simulink model "PMSM_FOC_R2026a"  (R2026a)
settings: Solver=ode4  StopTime=1  FixedStep=timing_h  MaxStep=1e-6
InitFcn:
  | % Embedded verbatim in the model InitFcn; no helper file is needed to run SLX.
  | teach_model = bdroot;
  | teach_workspace = get_param(teach_model,'ModelWorkspace');
  | teach_cfg_path = [teach_model '/时序设置'];
  | teach_divider = str2double(get_param(teach_cfg_path,'speed_divider'));
  | teach_cycles = str2double(get_param(teach_cfg_path,'pwm_cycles'));
  | validateattributes(teach_divider,{'double'},{'scalar','real','finite','integer','>=',1,'<=',1000});
  | validateattributes(teach_cycles,{'double'},{'scalar','real','finite','integer','>=',1,'<=',20});
  | teach_dt = getVariable(teach_workspace,'dt');
  | teach_period = getVariable(teach_workspace,'Ts_speed');
  | if strcmp(get_param(teach_cfg_path,'speed_on'),'on')
  |     teach_period = teach_dt*teach_divider;
  | end
  | assert(teach_period >= teach_dt && abs(teach_period/teach_dt-round(teach_period/teach_dt))<1e-9, ...
  |     '速度环周期必须为电流控制周期的正整数倍。');
  | teach_names = {'teaching_Ts_speed','teach_pwm_on','teach_pwm_cycles'};
  | teach_values_to_set = {teach_period,double(strcmp(get_param(teach_cfg_path,'pwm_on'),'on')),teach_cycles};
  | for teach_index = 1:numel(teach_names)
  |     if ~isequaln(getVariable(teach_workspace,teach_names{teach_index}),teach_values_to_set{teach_index})
  |         assignin(teach_workspace,teach_names{teach_index},teach_values_to_set{teach_index});
  |     end
  | end
  | 
  | 
  | assignin(get_param(bdroot,'ModelWorkspace'),'decoupling_enabled',double(strcmp(get_param([bdroot '/解耦'],'enabled'),'on')));
  | % Embedded in InitFcn after the pre-existing teaching initialization.
  | tim_m=bdroot;tim_ws=get_param(tim_m,'ModelWorkspace');tim_path=[tim_m '/时序设置'];
  | tim_on=double(strcmp(get_param(tim_path,'real_on'),'on'));
  | tim_period=getVariable(tim_ws,'dt');tim_speed=getVariable(tim_ws,'teaching_Ts_speed');
  | tim_trigger=str2double(get_param(tim_path,'trigger_us'))*1e-6;
  | tim_sync=str2double(get_param(tim_path,'sync_us'))*1e-6;
  | tim_compute=str2double(get_param(tim_path,'compute_us'))*1e-6;
  | tim_guard=str2double(get_param(tim_path,'settle_us'))*1e-6;
  | tim_window=double(strcmp(get_param(tim_path,'window_on'),'on'));
  | tim_hold=double(strcmp(get_param(tim_path,'invalid_hold_on'),'on'));
  | tim_mode=double(strcmp(get_param(tim_path,'update_mode'),'仅谷底（对照）'));
  | tim_h=1e-6;tim_control=tim_period;tim_speed_sample=tim_speed;
  | tim_static=-1;
  | tim_carrier=[0 tim_period/2 0];
  | validateattributes([tim_trigger tim_sync tim_compute tim_guard],{'double'},{'real','finite','nonnegative'});
  | if tim_on
  |  assert(strcmp(get_param(tim_path,'pwm_on'),'off'),'真实时序与旧整周期输出延迟不可同时启用。');
  |  assert(strcmp(get_param([tim_m '/采样设置'],'delay_on'),'off'),'真实时序与旧整周期采样延迟不可同时启用。');
  |  tim_h=62.5e-9;
  |  tim_grid_divider=str2double(get_param(tim_path,'grid_divider'));
  |  validateattributes(tim_grid_divider,{'double'},{'scalar','integer','>=',1,'<=',2});
  |  % Optional finer grid for convergence checks, still configured explicitly.
  |  tim_h=tim_h/tim_grid_divider;
  |  validateattributes(tim_h,{'double'},{'scalar','finite','positive'});
  |  tim_jeos=tim_trigger+tim_sync+4.5e-6;
  |  assert(tim_compute>=tim_h,'计算耗时至少为一个事件网格，避免写入读取同拍未完成指令。');
  |  assert(tim_jeos+tim_compute<tim_period,'本版要求整组转换及计算在同一PWM周期内完成。');
  |  assert(tim_jeos>0 && tim_jeos<tim_period);
  |  timing_grid_values=[tim_trigger tim_sync tim_compute tim_guard 1.1875e-6 1.5e-6 tim_period tim_speed];
  |  assert(all(abs(timing_grid_values/tim_h-round(timing_grid_values/tim_h))<1e-7),'事件时间必须落在62.5ns（或更细）网格上。');
  |  tim_control=[tim_period tim_jeos];
  |  tim_static=0;
  |  tim_speed_sample=[tim_speed tim_jeos+tim_speed-tim_period];
  |  % Existing comparator is carrier>=threshold; inverted carrier implements PWM1.
  |  tim_carrier=[tim_period/2 0 tim_period/2];
  | ... (+37 lines)
model workspace (MATLAB code in the model file):
  | % Embedded reference for the CHENSHA 200W nominal firmware profile.
  | % Source: AxDr_L dev 48d6e86814ac6657b1313b4c92ef24c88f492e07,
  | % User/config/motor_config.h. Not a measured plant identification.
  | % This script is embedded into the SLX Model Workspace; no path dependency.
  | T=1e-6; % Numerical step [s]; switching detail remains ideal/average equivalent
  | MotorProfile='CHENSHA 200W / firmware profile revision 2';
  | MotorSourceCommit='48d6e86814ac6657b1313b4c92ef24c88f492e07';
  | Pn=200; % Nameplate power [W], stored as specified; not forced to equal Tn*wm
  | Un=24; Vdc=24;
  | I_rated_rms=11.5; % Phase RMS [A], nameplate
  | I_peak_rms=23; % Phase RMS [A], nameplate peak
  | In=sqrt(2)*I_rated_rms; % Phase amplitude / dq nominal current [A]
  | I_peak=sqrt(2)*I_peak_rms; % Phase amplitude [A]
  | n=3000; % Speed reference and nominal speed [rpm]
  | p=5; % Pole pairs
  | Rs=0.105125; % Phase resistance [ohm], firmware profile convention
  | Ld=103.7615e-6; Lq=103.7615e-6; Ls=Ld; % dq inductance [H]
  | phis=0.06/(sqrt(2)*1.5*p); % Flux [Wb], derived from Kt_rms; Ke definition pending
  | J=32e-6; % Rotor inertia [kg*m^2], profile value; coupled inertia not identified
  | F=0; % Firmware profile placeholder; does not prove physical friction is zero
  | Kt=1.5*p*phis; % Torque per dq amplitude [N*m/A]
  | Tn=0.69; T_peak=1.38; % Nameplate torque [N*m]
  | Iq_limit=8; % Firmware bench command limit [A], not RMS nameplate current
  | accel_limit_rad_s2=1200; % Stored only; a command ramp is not implemented here
  | speed_peak_rad_s=335; % Stored only; speed protection is not implemented here
  | I_protection_A=10; Vbus_protection_high_V=30; Vbus_protection_low_V=10;
  | % Protection values above are references, not active trip logic in this model.
  | RE=10000; rr=2*pi/RE; % Mechanical counts/revolution; ABZ estimator not implemented
  | encoder_direction=-1; % Stored firmware setting; ideal plant angle stays unchanged
  | fN=p*n/60; wN=2*pi*fN;
  | ki_p=0.8; ki_i=1; % Original unused/auxiliary constants retained
  | fc=20e3; Ts=1/fc; dt=Ts;
  | Ts_speed=2*dt; % Base speed task 10kHz; current/PWM 20kHz
  | w_sb=2*pi*fN*1.2;
  | fcb=1000; fwb=50; wc=2*pi*fcb; wsc=2*pi*fwb;
  | % fcb/fwb describe the previous gain design, not measured bandwidth of this motor.
  | K=30/pi; % Mechanical rad/s to rpm
  | % PI_GAINS_FROZEN: inserted from the validated previous workspace, bit-for-bit.
  | kp_w=0.00069087230807625508;
  | ki_w=0.04340878735241975;
  | ks_w=0.98718608264211138;
  | kp_id=0.7539822368615503;
  | ki_id=879.64594300514204;
  | ks_id=1.1309733552923253;
  | kp_iq=0.7539822368615503;
  | ki_iq=879.64594300514204;
  | ks_iq=1.1309733552923253;
  | Bm=0;
  | uplimit_w=Kt*Iq_limit; downlimit_w=-uplimit_w; % Speed PI output is torque [N*m]
  | % Ld=Lq and id_ref=0, so Te_ref/Kt is exactly the iq demand before dynamics.
  | uplimit_id=Vdc/sqrt(3); downlimit_id=-uplimit_id;
  | uplimit_iq=Vdc/sqrt(3); downlimit_iq=-uplimit_iq;
  | teaching_Ts_speed=Ts_speed; teach_pwm_on=0; teach_pwm_cycles=1;
  | 
  | decoupling_enabled=1; voltage_utilization=0.96; % Algorithm stage 2; PI gains frozen
  | 
  | timing_on=0; timing_h=1e-6; timing_control_sample=dt; timing_speed_sample=Ts_speed; timing_static_math=-1;
  | timing_carrier_y=[0 Ts/2 0];
  | timing_adc_cfg=[0 0 0 1e-6 Ts 24.375e-6 1.1875e-6 1.5e-6 0 .5e-6 2];
  | timing_pwm_cfg=[0 1e-6 Ts 24.375e-6 1.1875e-6 1.5e-6 0 5e-6 0 4000];
  | 
  | dead_gate_on=0; dead_h=1e-6; dead_gate_cfg=[0 1e-6 .5e-6];
  | dead_comp_cfg=[0 .5e-6 Ts .05]; dead_bridge_cfg=[p phis .01 0 .01 .7];
undefined symbols (not defined in the file or in its folder): DiscIntNeverNeededParam
libraries: simulink x3
(part 2 of 2)

== system PMSM_FOC_R2026a/功率观测 ==
  note: 01 理想相电压 [V]
  note: 02 实际相电压 [V]
  note: 03 平均压降 [V]
  实际相电压 : Scope
      settings: SampleTime=T  Title=实际相电压 [V]
  平均压降 : Scope
      settings: SampleTime=dt  Title=平均压降 [V]
  总览 : Scope  NumInputPorts=8
      settings: SampleTime=T  TimeSpan=0.12  ActiveDisplayString=8  Title=dq补偿 [V]
  极性保留 : Terminator
  理想相电压 : Scope
      settings: SampleTime=T  Title=理想相电压 [V]
  真实电流保留 : Terminator
  续流分组 : Demux  Outputs=[3 3 3]
  补偿分组 : Demux  Outputs=[3 2 3]
  wires:
  [ObsPhaseIdeal] -> 理想相电压/1, 总览/1
  [ObsPhaseActual] -> 实际相电压/1, 总览/2
  [ObsPowerDrop] -> 平均压降/1, 总览/3
  [ObsFreewheel] -> 续流分组/1
  续流分组/3 -> 真实电流保留/1
  [ObsDeadComp] -> 补偿分组/1
  补偿分组/3 -> 极性保留/1
  [SWact] -> 总览/4
  续流分组/1 -> 总览/5
  续流分组/2 -> 总览/6
  补偿分组/1 -> 总览/7
  补偿分组/2 -> 总览/8

== system PMSM_FOC_R2026a/功率设置 ==
  三相压降 : Mux  Inputs=3
  压降1 : Fcn  Expr=dead_on*dead_us*1e-6/Ts*(u(4)+drop_on*vf)*u(1)/(abs(u(1))+blend_A)+drop_on*ron*u(1)
  压降2 : Fcn  Expr=dead_on*dead_us*1e-6/Ts*(u(4)+drop_on*vf)*u(2)/(abs(u(2))+blend_A)+drop_on*ron*u(2)
  压降3 : Fcn  Expr=dead_on*dead_us*1e-6/Ts*(u(4)+drop_on*vf)*u(3)/(abs(u(3))+blend_A)+drop_on*ron*u(3)
  去共模 : Gain  Gain=eye(3)-ones(3)/3  Multiplication=Matrix(K*u)
  启用 : Constant  Value=(~dead_gate_on)&&(dead_on||drop_on)
  周期电流 : ZeroOrderHold  SampleTime=Ts
  记录_obs_power_drop : ToWorkspace  VariableName=obs_power_drop  SaveFormat=Timeseries  SampleTime=timing_control_sample
  输入 : Mux  Inputs=2
  tag scope: ObsPowerDrop=global, ObsPowerOn=global
  wires:
  [Currentabc] -> 周期电流/1
  周期电流/1 -> 输入/1
  [UDC] -> 输入/2
  输入/1 -> 压降1/1, 压降2/1, 压降3/1
  压降1/1 -> 三相压降/1
  压降2/1 -> 三相压降/2
  压降3/1 -> 三相压降/3
  三相压降/1 -> 去共模/1
  去共模/1 -> [ObsPowerDrop], 记录_obs_power_drop/1
  启用/1 -> [ObsPowerOn]

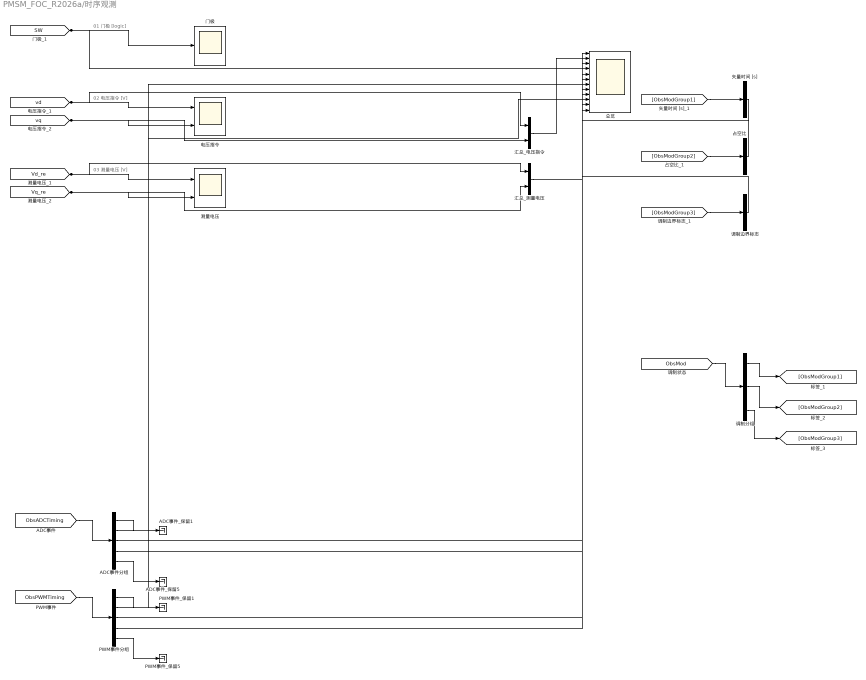
== system PMSM_FOC_R2026a/时序观测 ==
  note: 01 门极 [logic]
  note: 02 电压指令 [V]
  note: 03 测量电压 [V]
  ADC事件_保留1 : Terminator
  ADC事件_保留5 : Terminator
  ADC事件分组 : Demux  Outputs=[1 5 3 4 2]
  PWM事件_保留1 : Terminator
  PWM事件_保留5 : Terminator
  PWM事件分组 : Demux  Outputs=[2 3 3 1 3]
  占空比 : Mux  Inputs=1
  总览 : Scope  NumInputPorts=12
      settings: SampleTime=T  TimeSpan=0.12  ActiveDisplayString=12  Title=采样至生效 [s]
  汇总_测量电压 : Mux  Inputs=2
  汇总_电压指令 : Mux  Inputs=2
  测量电压 : Scope  NumInputPorts=2
      settings: SampleTime=T  Title=测量电压 [V]
  电压指令 : Scope  NumInputPorts=2
      settings: SampleTime=dt  Title=电压指令 [V]
  矢量时间 [s] : Mux  Inputs=1
  调制分组 : Demux  Outputs=[3 3 2]
  调制边界标志 : Mux  Inputs=1
  门极 : Scope
      settings: SampleTime=T  Title=门极 [logic]
  wires:
  [SW] -> 门极/1, 总览/1
  [vd] -> 电压指令/1, 汇总_电压指令/1
  [vq] -> 电压指令/2, 汇总_电压指令/2
  [Vd_re] -> 测量电压/1, 汇总_测量电压/1
  [Vq_re] -> 测量电压/2, 汇总_测量电压/2
  汇总_电压指令/1 -> 总览/2
  汇总_测量电压/1 -> 总览/3
  [ObsMod] -> 调制分组/1
  调制分组/1 -> [ObsModGroup1]
  调制分组/2 -> [ObsModGroup2]
  调制分组/3 -> [ObsModGroup3]
  [ObsModGroup1] -> 矢量时间 [s]/1
  矢量时间 [s]/1 -> 总览/4
  [ObsModGroup2] -> 占空比/1
  占空比/1 -> 总览/5
  [ObsModGroup3] -> 调制边界标志/1
  调制边界标志/1 -> 总览/6
  [ObsADCTiming] -> ADC事件分组/1
  ADC事件分组/1 -> ADC事件_保留1/1
  ADC事件分组/5 -> ADC事件_保留5/1
  [ObsPWMTiming] -> PWM事件分组/1
  PWM事件分组/1 -> PWM事件_保留1/1
  PWM事件分组/5 -> PWM事件_保留5/1
  ADC事件分组/2 -> 总览/7
  ADC事件分组/3 -> 总览/8
  ADC事件分组/4 -> 总览/9
  PWM事件分组/2 -> 总览/10
  PWM事件分组/3 -> 总览/11
  PWM事件分组/4 -> 总览/12

== system PMSM_FOC_R2026a/时序设置 ==

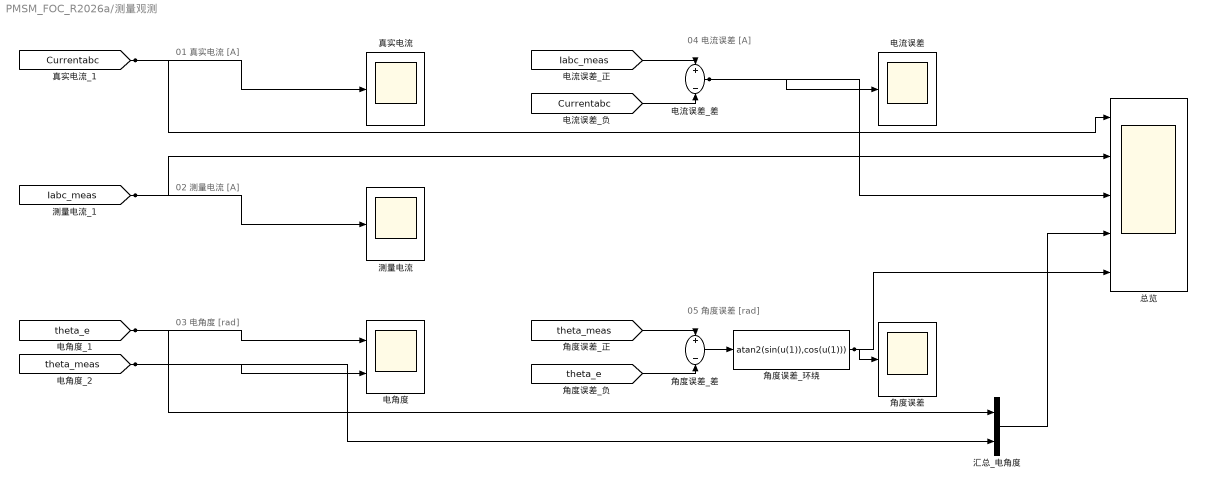
== system PMSM_FOC_R2026a/测量观测 ==
  note: 01 真实电流 [A]
  note: 02 测量电流 [A]
  note: 03 电角度 [rad]
  note: 04 电流误差 [A]
  note: 05 角度误差 [rad]
  总览 : Scope  NumInputPorts=5
      settings: SampleTime=dt  TimeSpan=0.12  ActiveDisplayString=5  Title=角度误差 [rad]
  汇总_电角度 : Mux  Inputs=2
  测量电流 : Scope
      settings: SampleTime=dt  Title=测量电流 [A]
  电流误差 : Scope
      settings: SampleTime=dt  Title=电流误差 [A]
  电流误差_差 : Sum  Inputs=+-
  电角度 : Scope  NumInputPorts=2
      settings: SampleTime=dt  Title=电角度 [rad]
  真实电流 : Scope
      settings: SampleTime=dt  Title=真实电流 [A]
  角度误差 : Scope
      settings: SampleTime=dt  Title=角度误差 [rad]
  角度误差_差 : Sum  Inputs=+-
  角度误差_环绕 : Fcn  Expr=atan2(sin(u(1)),cos(u(1)))
  wires:
  [Currentabc] -> 真实电流/1, 总览/1
  [Iabc_meas] -> 测量电流/1, 总览/2
  [theta_e] -> 电角度/1, 汇总_电角度/1
  [theta_meas] -> 电角度/2, 汇总_电角度/2
  [Iabc_meas] -> 电流误差_差/1
  [Currentabc] -> 电流误差_差/2
  电流误差_差/1 -> 电流误差/1, 总览/3
  [theta_meas] -> 角度误差_差/1
  [theta_e] -> 角度误差_差/2
  角度误差_差/1 -> 角度误差_环绕/1
  角度误差_环绕/1 -> 角度误差/1, 总览/5
  汇总_电角度/1 -> 总览/4

== system PMSM_FOC_R2026a/角度设置 ==
  传递延迟 : Delay  DelayLength=delay_cycles  InitialCondition=0  SampleTime=timing_control_sample
  偏置 : Constant  Value=bias_on*bias_deg*pi/180
  偏置求和 : Sum
  启用 : Constant  Value=bias_on||quant_on||delay_on
  延迟开关 : Constant  Value=delay_on
  延迟选择 : Switch  Criteria=u2 ~= 0  SaturateOnIntegerOverflow=off  InputSameDT=off
  总选择 : Switch  Criteria=u2 ~= 0  SaturateOnIntegerOverflow=off  InputSameDT=off
  最短角差 : Fcn  Expr=atan2(sin(u(1)),cos(u(1)))
  角度差 : Sum  Inputs=+-
  角度环绕 : Fcn  Expr=u(1)-2*pi*floor(u(1)/(2*pi))
  记录_log_theta_error : ToWorkspace  VariableName=log_theta_error  SaveFormat=Timeseries  SampleTime=timing_control_sample
  记录_log_theta_meas : ToWorkspace  VariableName=log_theta_meas  SaveFormat=Timeseries  SampleTime=timing_control_sample
  记录_log_theta_true : ToWorkspace  VariableName=log_theta_true  SaveFormat=Timeseries  SampleTime=timing_control_sample
  量化 : Quantizer  QuantizationInterval=step_deg*pi/180
  量化开关 : Constant  Value=quant_on
  量化选择 : Switch  Criteria=u2 ~= 0  SaturateOnIntegerOverflow=off  InputSameDT=off
  tag scope: theta_meas=global
  wires:
  [theta_e] -> 偏置求和/1, 总选择/3, 角度差/2, 记录_log_theta_true/1
  偏置/1 -> 偏置求和/2
  偏置求和/1 -> 量化/1, 量化选择/3
  量化/1 -> 量化选择/1
  量化开关/1 -> 量化选择/2
  量化选择/1 -> 角度环绕/1
  角度环绕/1 -> 传递延迟/1, 延迟选择/3
  传递延迟/1 -> 延迟选择/1
  延迟开关/1 -> 延迟选择/2
  延迟选择/1 -> 总选择/1
  启用/1 -> 总选择/2
  总选择/1 -> [theta_meas], 角度差/1, 记录_log_theta_meas/1
  角度差/1 -> 最短角差/1
  最短角差/1 -> 记录_log_theta_error/1

== system PMSM_FOC_R2026a/解耦 ==

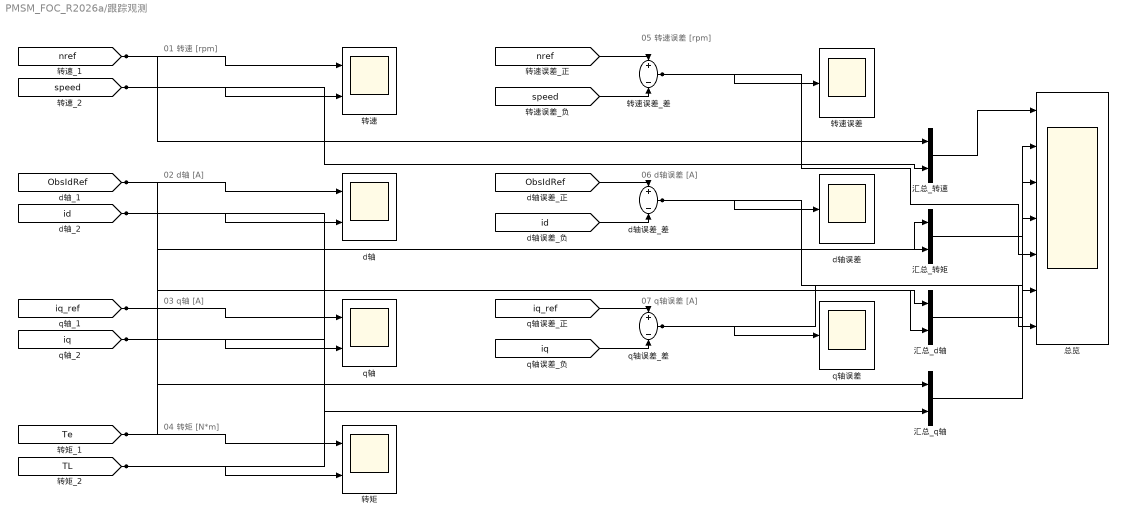
== system PMSM_FOC_R2026a/跟踪观测 ==
  note: 01 转速 [rpm]
  note: 02 d轴 [A]
  note: 03 q轴 [A]
  note: 04 转矩 [N*m]
  note: 05 转速误差 [rpm]
  note: 06 d轴误差 [A]
  note: 07 q轴误差 [A]
  d轴 : Scope  NumInputPorts=2
      settings: SampleTime=dt  Title=d轴 [A]
  d轴误差 : Scope
      settings: SampleTime=dt  Title=d轴误差 [A]
  d轴误差_差 : Sum  Inputs=+-
  q轴 : Scope  NumInputPorts=2
      settings: SampleTime=dt  Title=q轴 [A]
  q轴误差 : Scope
      settings: SampleTime=dt  Title=q轴误差 [A]
  q轴误差_差 : Sum  Inputs=+-
  总览 : Scope  NumInputPorts=7
      settings: SampleTime=dt  TimeSpan=0.12  ActiveDisplayString=7  Title=q轴误差 [A]
  汇总_d轴 : Mux  Inputs=2
  汇总_q轴 : Mux  Inputs=2
  汇总_转矩 : Mux  Inputs=2
  汇总_转速 : Mux  Inputs=2
  转矩 : Scope  NumInputPorts=2
      settings: SampleTime=dt  Title=转矩 [N*m]
  转速 : Scope  NumInputPorts=2
      settings: SampleTime=dt  Title=转速 [rpm]
  转速误差 : Scope
      settings: SampleTime=dt  Title=转速误差 [rpm]
  转速误差_差 : Sum  Inputs=+-
  wires:
  [nref] -> 转速/1, 汇总_转速/1
  [speed] -> 转速/2, 汇总_转速/2
  [ObsIdRef] -> d轴/1, 汇总_d轴/1
  [id] -> d轴/2, 汇总_d轴/2
  [iq_ref] -> q轴/1, 汇总_q轴/1
  [iq] -> q轴/2, 汇总_q轴/2
  [Te] -> 转矩/1, 汇总_转矩/1
  [TL] -> 转矩/2, 汇总_转矩/2
  [nref] -> 转速误差_差/1
  [speed] -> 转速误差_差/2
  转速误差_差/1 -> 转速误差/1, 总览/5
  [ObsIdRef] -> d轴误差_差/1
  [id] -> d轴误差_差/2
  d轴误差_差/1 -> d轴误差/1, 总览/6
  [iq_ref] -> q轴误差_差/1
  [iq] -> q轴误差_差/2
  q轴误差_差/1 -> q轴误差/1, 总览/7
  汇总_转速/1 -> 总览/1
  汇总_转矩/1 -> 总览/2
  汇总_d轴/1 -> 总览/3
  汇总_q轴/1 -> 总览/4

== system PMSM_FOC_R2026a/输出延迟 ==
  指令 : Inport
  CCR预装载 : MATLAB Function  TreatAsAtomicUnit=on
  事件时钟 : DigitalClock  SampleTime=timing_h
  启用 : Constant  Value=teach_pwm_on
  周期延迟 : Delay  DelayLength=teach_pwm_cycles  InitialCondition=0  SampleTime=timing_control_sample
  指令缓存 : UnitDelay  InitialCondition=Ts/4  SampleTime=timing_h
  时序参数 : Constant  Value=timing_pwm_cfg
  记录_log_Tcm_applied : ToWorkspace  VariableName=log_Tcm_applied  SaveFormat=Timeseries  SampleTime=timing_control_sample
  记录_log_Tcm_requested : ToWorkspace  VariableName=log_Tcm_requested  SaveFormat=Timeseries  SampleTime=timing_control_sample
  记录_obs_pwm_timing : ToWorkspace  VariableName=obs_pwm_timing  SaveFormat=Timeseries  SampleTime=timing_h
  输出方式 : VariantSource  VariantControls={real_mode==1, real_mode==0}
  选择 : Switch  Criteria=u2 ~= 0  SaturateOnIntegerOverflow=off  InputSameDT=off
  阈值向量 : Reshape
  生效 : Outport
  tag scope: ObsPWMTiming=global
  wires:
  指令/1 -> 周期延迟/1, 选择/3, 记录_log_Tcm_requested/1, 指令缓存/1
  周期延迟/1 -> 选择/1
  启用/1 -> 选择/2
  选择/1 -> 输出方式/2
  事件时钟/1 -> CCR预装载/1(t)
  时序参数/1 -> CCR预装载/3(cfg)
  指令缓存/1 -> CCR预装载/2(request)
  CCR预装载/1(applied) -> 阈值向量/1
  输出方式/1 -> 生效/1, 记录_log_Tcm_applied/1
  阈值向量/1 -> 输出方式/1
  CCR预装载/2(diag) -> 记录_obs_pwm_timing/1, [ObsPWMTiming]

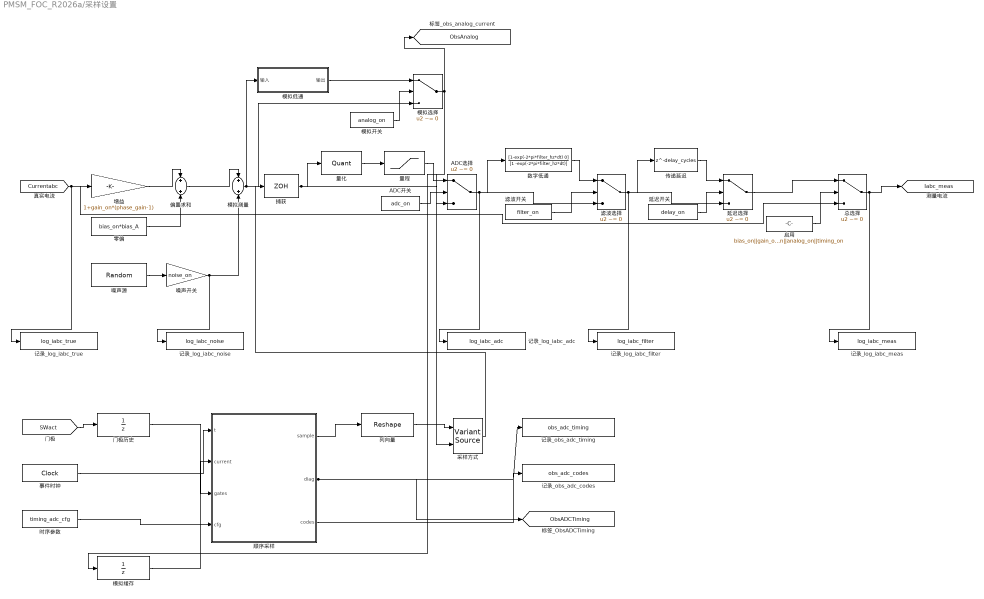
== system PMSM_FOC_R2026a/采样设置 ==
  ADC开关 : Constant  Value=adc_on
  ADC选择 : Switch  Criteria=u2 ~= 0  SaturateOnIntegerOverflow=off  InputSameDT=off
  事件时钟 : DigitalClock  SampleTime=timing_h
  传递延迟 : Delay  DelayLength=delay_cycles  InitialCondition=0  SampleTime=timing_control_sample
  偏置求和 : Sum
  列向量 : Reshape  OutputDimensionality=Column vector (2-D)
  启用 : Constant  Value=bias_on||gain_on||noise_on||adc_on||filter_on||delay_on||analog_on||timing_on
  噪声开关 : Gain  Gain=noise_on
  噪声源 : RandomNumber  Mean=[0 0 0]  Variance=noise_rms^2  Seed=noise_seed+[0 1 2]  SampleTime=timing_control_sample
  增益 : Gain  Gain=1+gain_on*(phase_gain-1)
  延迟开关 : Constant  Value=delay_on
  延迟选择 : Switch  Criteria=u2 ~= 0  SaturateOnIntegerOverflow=off  InputSameDT=off
  总选择 : Switch  Criteria=u2 ~= 0  SaturateOnIntegerOverflow=off  InputSameDT=off
  捕获 : ZeroOrderHold  SampleTime=timing_control_sample
  数字低通 : DiscreteTransferFcn  Numerator=[1-exp(-2*pi*filter_hz*dt) 0]  Denominator=[1 -exp(-2*pi*filter_hz*dt)]  SampleTime=timing_control_sample
  时序参数 : Constant  Value=timing_adc_cfg
  模拟低通 : Subsystem
  模拟开关 : Constant  Value=analog_on
  模拟测量 : Sum
  模拟缓存 : UnitDelay  InitialCondition=[0;0;0]  SampleTime=timing_h
  模拟选择 : Switch  Criteria=u2 ~= 0  SaturateOnIntegerOverflow=off  InputSameDT=off
  滤波开关 : Constant  Value=filter_on
  滤波选择 : Switch  Criteria=u2 ~= 0  SaturateOnIntegerOverflow=off  InputSameDT=off
  记录_log_iabc_adc : ToWorkspace  VariableName=log_iabc_adc  SaveFormat=Timeseries  SampleTime=timing_control_sample
  记录_log_iabc_filter : ToWorkspace  VariableName=log_iabc_filter  SaveFormat=Timeseries  SampleTime=timing_control_sample
  记录_log_iabc_meas : ToWorkspace  VariableName=log_iabc_meas  SaveFormat=Timeseries  SampleTime=timing_control_sample
  记录_log_iabc_noise : ToWorkspace  VariableName=log_iabc_noise  SaveFormat=Timeseries  SampleTime=timing_control_sample
  记录_log_iabc_true : ToWorkspace  VariableName=log_iabc_true  SaveFormat=Timeseries  SampleTime=timing_control_sample
  记录_obs_adc_codes : ToWorkspace  VariableName=obs_adc_codes  SaveFormat=Timeseries  SampleTime=timing_control_sample
  记录_obs_adc_timing : ToWorkspace  VariableName=obs_adc_timing  SaveFormat=Timeseries  SampleTime=timing_h
  采样方式 : VariantSource  VariantControls={real_mode==1, real_mode==0}
  量化 : Quantizer  QuantizationInterval=2*adc_span/2^adc_bits
  量程 : Saturate  UpperLimit=adc_span-2*adc_span/2^adc_bits  LowerLimit=-adc_span
  门极历史 : UnitDelay  InitialCondition=[0 1 0 1 0 1]  SampleTime=timing_h
  零偏 : Constant  Value=bias_on*bias_A
  顺序采样 : MATLAB Function  TreatAsAtomicUnit=on
  tag scope: Iabc_meas=global, ObsADCTiming=global, ObsAnalog=global
  wires:
  [Currentabc] -> 增益/1, 总选择/3, 记录_log_iabc_true/1
  增益/1 -> 偏置求和/1
  零偏/1 -> 偏置求和/2
  偏置求和/1 -> 模拟测量/1
  噪声源/1 -> 噪声开关/1
  噪声开关/1 -> 模拟测量/2, 记录_log_iabc_noise/1
  捕获/1 -> 量化/1, ADC选择/3
  量化/1 -> 量程/1
  量程/1 -> ADC选择/1
  ADC开关/1 -> ADC选择/2
  ADC选择/1 -> 数字低通/1, 滤波选择/3, 记录_log_iabc_adc/1
  数字低通/1 -> 滤波选择/1
  滤波开关/1 -> 滤波选择/2
  滤波选择/1 -> 传递延迟/1, 延迟选择/3, 记录_log_iabc_filter/1
  传递延迟/1 -> 延迟选择/1
  延迟开关/1 -> 延迟选择/2
  延迟选择/1 -> 总选择/1
  启用/1 -> 总选择/2
  总选择/1 -> [Iabc_meas], 记录_log_iabc_meas/1
  模拟测量/1 -> 模拟低通/1(输入), 模拟选择/3
  模拟低通/1(输出) -> 模拟选择/1
  模拟开关/1 -> 模拟选择/2
  模拟选择/1 -> [ObsAnalog], 模拟缓存/1, 采样方式/2
  [SWact] -> 门极历史/1
  事件时钟/1 -> 顺序采样/1(t)
  门极历史/1 -> 顺序采样/3(gates)
  时序参数/1 -> 顺序采样/4(cfg)
  模拟缓存/1 -> 顺序采样/2(current)
  顺序采样/1(sample) -> 列向量/1
  采样方式/1 -> 捕获/1
  列向量/1 -> 采样方式/1
  顺序采样/2(diag) -> 记录_obs_adc_timing/1, [ObsADCTiming]
  顺序采样/3(codes) -> 记录_obs_adc_codes/1

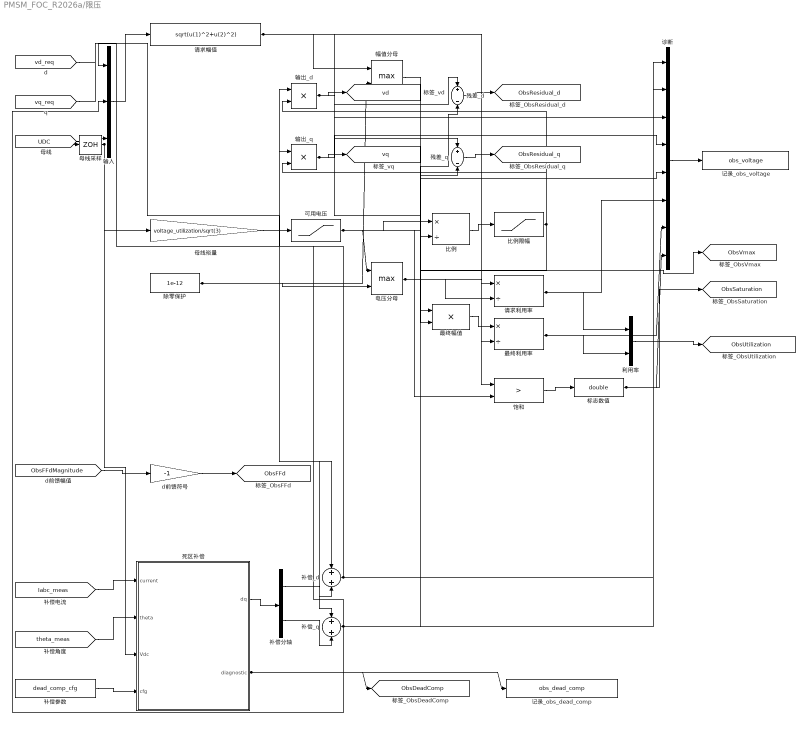
== system PMSM_FOC_R2026a/限压 ==
  d前馈符号 : Gain  Gain=-1
  利用率 : Mux  Inputs=2
  可用电压 : Saturate  UpperLimit=inf  LowerLimit=0
  幅值分母 : MinMax  Function=max  Inputs=2
  最终利用率 : Product  Inputs=*/
  最终幅值 : Product
  标志数值 : DataTypeConversion  OutDataTypeStr=double  SaturateOnIntegerOverflow=off  RndMeth=Floor
  死区补偿 : MATLAB Function  TreatAsAtomicUnit=on
  残差_d : Sum  Inputs=+-
  残差_q : Sum  Inputs=+-
  母线裕量 : Gain  Gain=voltage_utilization/sqrt(3)
  母线采样 : ZeroOrderHold  SampleTime=timing_control_sample
  比例 : Product  Inputs=*/
  比例限幅 : Saturate  UpperLimit=1  LowerLimit=0
  电压分母 : MinMax  Function=max  Inputs=2
  补偿_d : Sum
  补偿_q : Sum
  补偿分轴 : Demux  Outputs=2
  补偿参数 : Constant  Value=dead_comp_cfg
  记录_obs_dead_comp : ToWorkspace  VariableName=obs_dead_comp  SaveFormat=Timeseries  SampleTime=timing_control_sample
  记录_obs_voltage : ToWorkspace  VariableName=obs_voltage  SaveFormat=Timeseries  SampleTime=timing_control_sample
  诊断 : Mux  Inputs=8
  请求利用率 : Product  Inputs=*/
  请求幅值 : Fcn  Expr=sqrt(u(1)^2+u(2)^2)
  输入 : Mux  Inputs=3
  输出_d : Product
  输出_q : Product
  除零保护 : Constant  Value=1e-12
  饱和 : RelationalOperator  Operator=>  OutDataTypeStr=boolean  RndMeth=Simplest  InputSameDT=off
  tag scope: ObsDeadComp=global, ObsFFd=global, ObsResidual_d=global, ObsResidual_q=global, ObsSaturation=global, ObsUtilization=global, ObsVmax=global, vd=global, vq=global
  wires:
  [UDC] -> 母线采样/1
  [vd_req] -> 补偿_d/1
  [vq_req] -> 补偿_q/1
  母线采样/1 -> 输入/3, 母线裕量/1, 死区补偿/3(Vdc)
  输入/1 -> 请求幅值/1
  母线裕量/1 -> 可用电压/1
  请求幅值/1 -> 幅值分母/1, 请求利用率/1, 最终幅值/1, 饱和/1
  除零保护/1 -> 幅值分母/2, 电压分母/2
  可用电压/1 -> 电压分母/1, 比例/1, 诊断/5, 饱和/2, [ObsVmax]
  幅值分母/1 -> 比例/2
  比例/1 -> 比例限幅/1
  比例限幅/1 -> 输出_d/2, 输出_q/2, 最终幅值/2
  输出_d/1 -> [vd], 残差_d/1, 诊断/3
  残差_d/1 -> [ObsResidual_d]
  输出_q/1 -> [vq], 残差_q/1, 诊断/4
  残差_q/1 -> [ObsResidual_q]
  电压分母/1 -> 请求利用率/2, 最终利用率/2
  请求利用率/1 -> 诊断/6, 利用率/1
  最终幅值/1 -> 最终利用率/1
  最终利用率/1 -> 诊断/7, 利用率/2
  饱和/1 -> 标志数值/1
  标志数值/1 -> 诊断/8, [ObsSaturation]
  诊断/1 -> 记录_obs_voltage/1
  利用率/1 -> [ObsUtilization]
  [ObsFFdMagnitude] -> d前馈符号/1
  d前馈符号/1 -> [ObsFFd]
  [Iabc_meas] -> 死区补偿/1(current)
  [theta_meas] -> 死区补偿/2(theta)
  补偿参数/1 -> 死区补偿/4(cfg)
  死区补偿/1(dq) -> 补偿分轴/1
  补偿分轴/1 -> 补偿_d/2
  补偿_d/1 -> 输入/1, 输出_d/1, 残差_d/2, 诊断/1
  补偿分轴/2 -> 补偿_q/2
  补偿_q/1 -> 输入/2, 输出_q/1, 残差_q/2, 诊断/2
  死区补偿/2(diagnostic) -> [ObsDeadComp], 记录_obs_dead_comp/1

== system PMSM_FOC_R2026a/采样设置/模拟低通 ==
  输入 : Inport
  RC1 : TransferFcn  Numerator=[2*pi*analog_hz]  Denominator=[1 2*pi*analog_hz]
  RC2 : TransferFcn  Numerator=[2*pi*analog_hz]  Denominator=[1 2*pi*analog_hz]
  RC3 : TransferFcn  Numerator=[2*pi*analog_hz]  Denominator=[1 2*pi*analog_hz]
  分相 : Demux  Outputs=3
  合相 : Mux  Inputs=3
  输出 : Outport
  wires:
  输入/1 -> 分相/1
  合相/1 -> 输出/1
  分相/1 -> RC1/1
  RC1/1 -> 合相/1
  分相/2 -> RC2/1
  RC2/1 -> 合相/2
  分相/3 -> RC3/1
  RC3/1 -> 合相/3

== matlab function PMSM_FOC_R2026a/采样设置/顺序采样 ==
  settings: updateMethod=DISCRETE  sampleTime=timing_h
  data: t input; sample output size=[1 3]; current input; gates input; cfg input; diag output size=[1 15]; codes output size=[1 3]
function [sample,diag,codes] = timing_adc(t,current,gates,cfg)
%#codegen
% cfg: on, window, hold-invalid, h, Ts, trigger, aperture, rank, sync, guard, speed divider.
% Quantized event grid; outputs are published together at JEOS, in A/B/C order.
persistent captured delivered valid elapsed aperture_ok last_good raw_codes
if isempty(captured)
 captured=zeros(1,3);delivered=zeros(1,3);valid=zeros(1,3);
 elapsed=zeros(1,3);aperture_ok=ones(1,3);last_good=zeros(1,3);raw_codes=2048*ones(1,3);
end
sample=delivered;codes=raw_codes;diag=zeros(1,15);
if cfg(1)==0,return;end
h=cfg(4);N=round(cfg(5)/h);tick=round(t/h);phase=mod(tick,N);
tr=round((cfg(6)+cfg(9))/h);ap=round(cfg(7)/h);rank=round(cfg(8)/h);
guard=ceil(cfg(10)/h);pulse=zeros(1,5);
if phase==tr,pulse(1)=1;end
for k=1:3
 % Gates are sampled one grid tick earlier to avoid an algebraic gate loop.
 if gates(2*k)>0.5,elapsed(k)=elapsed(k)+1;else,elapsed(k)=0;end
 r=3-k;start=tr+r*rank;finish=start+ap;
 if phase==start,aperture_ok(k)=double(elapsed(k)>guard);end
 if phase>=start && phase<=finish && elapsed(k)<=guard,aperture_ok(k)=0;end
 if phase==finish
  valid(k)=aperture_ok(k);pulse(r+2)=1;
 end
 % Input read buffer is one tick old. Read on the following tick so the
 % captured physical value remains exactly at the aperture endpoint.
 if phase==finish+1
  captured(k)=current(k);
  % Low-side OFF has no phase-current observation. Zero is an explicit
  % teaching approximation, not a calibrated amplifier switching transient.
  if cfg(2)>0 && valid(k)==0,captured(k)=0;end
  if valid(k)>0,last_good(k)=captured(k);end
  if cfg(2)>0 && cfg(3)>0 && valid(k)==0,captured(k)=last_good(k);end
 end
end
jeos=tr+3*rank;
if phase==jeos
 delivered=captured;raw_codes=min(4095,max(0,round(2048+captured/(165/4096))));pulse(5)=1;
end
sample=delivered;codes=raw_codes;
% Phase, trigger, C/B/A hold pulses, JEOS, validity ABC, sampled ABC, sum.
diag=[phase*h pulse(1:4) pulse(5) valid delivered sum(delivered) ...
       double(mod(floor(tick/N),cfg(11))==cfg(11)-1 && phase==jeos) double(phase==jeos)];
end

== matlab function PMSM_FOC_R2026a/SVPWM Function v1.0 ==
  data: alpha input; beta input; Vdc input; Ts input; Tcm output; sector output; diagnostic output
function [Tcm,sector,diagnostic] = fcn(alpha,beta,Vdc,Ts)
% Original six-sector construction, with simultaneous overmodulation scaling.
% Tcm is a threshold in [0,Ts/2]; upper duty = 1-2*Tcm/Ts.
% diagnostic: t1,t2,total zero-vector time,Da,Db,Dc,overmodulated,bounds_guard.
Tcm=ones(1,3)*Ts/4;sector=0;
diagnostic=[0 0 Ts .5 .5 .5 0 0];
if Vdc<=0 || Ts<=0 || (alpha==0 && beta==0),return;end
ref1=beta;ref2=(-beta+sqrt(3)*alpha)/2;ref3=(-beta-sqrt(3)*alpha)/2;
sector=4*double(ref3>0)+2*double(ref2>0)+double(ref1>0);
X=Ts*sqrt(3)/Vdc*beta;
Y=Ts*sqrt(3)/Vdc*(sqrt(3)*alpha+beta)/2;
Z=Ts*sqrt(3)/Vdc*(-sqrt(3)*alpha+beta)/2;
switch sector
 case 1,t1=Z;t2=Y;
 case 2,t1=Y;t2=-X;
 case 3,t1=-Z;t2=X;
 case 4,t1=-X;t2=Z;
 case 5,t1=X;t2=-Y;
 otherwise,t1=-Y;t2=-Z;
end
t1=max(0,t1);t2=max(0,t2);
total=t1+t2;over=double(total>Ts);
if total>Ts
 scale=Ts/total;t1=t1*scale;t2=t2*scale;
end
tzero=max(0,Ts-t1-t2);
ta=tzero/4;tb=ta+t1/2;tc=tb+t2/2;
switch sector
 case 1,Tcm=[tb ta tc];
 case 2,Tcm=[ta tc tb];
 case 3,Tcm=[ta tb tc];
 case 4,Tcm=[tc tb ta];
 case 5,Tcm=[tc ta tb];
 case 6,Tcm=[tb tc ta];
end
guard=double(any(Tcm<-1e-12) || any(Tcm>Ts/2+1e-12));
Tcm=min(Ts/2,max(0,Tcm));
diagnostic=[t1 t2 tzero 1-2*Tcm/Ts over guard];
end

== matlab function PMSM_FOC_R2026a/输出延迟/CCR预装载 ==
  settings: updateMethod=DISCRETE  sampleTime=timing_h
  data: t input; applied output size=[1 3]; request input; cfg input; diag output size=[1 12]
function [applied,diag] = timing_pwm(t,request,cfg)
%#codegen
% cfg: on, h, Ts, trigger, aperture, rank, sync, compute, update mode, ARR.
% mode=0: RCR=0 update at both extrema; mode=1: underflow-only comparison.
% If a write coincides with UEV, UEV wins and the new CCR waits for the next UEV.
persistent shadow active pending shadow_seq active_seq writes stamp delay
if isempty(shadow)
 shadow=cfg(3)/4*ones(1,3);active=shadow;pending=false;
 shadow_seq=0;active_seq=0;writes=0;stamp=0;delay=0;
end
applied=active;diag=zeros(1,12);
if cfg(1)==0,return;end
h=cfg(2);N=round(cfg(3)/h);tick=round(t/h);phase=mod(tick,N);
jeos=round((cfg(4)+cfg(7)+3*cfg(6))/h);wr=jeos+round(cfg(8)/h);
update=(phase==0 || (cfg(9)==0 && phase==N/2));write=(phase==wr);
latched=false;
if update && pending
 active=shadow;active_seq=shadow_seq;pending=false;latched=true;delay=t-stamp;
end
if write
 duty=max(0,min(1,1-2*reshape(request,1,3)/cfg(3)));
 ccr=floor(duty*cfg(10)+1e-9);
 shadow=cfg(3)/2*(1-ccr/cfg(10));shadow_seq=shadow_seq+1;
 writes=writes+1;pending=true;stamp=floor(tick/N)*cfg(3)+jeos*h;
end
applied=active;
cnt=2*min(phase,N-phase)/N*cfg(10);
diag=[cnt double(phase>=N/2) double(update) double(write) double(latched) ...
 shadow_seq active_seq double(pending) delay shadow];
end

== matlab function PMSM_FOC_R2026a/Universal Bridge/门极死区 ==
  settings: updateMethod=DISCRETE  sampleTime=dead_h
  data: t input; gates output size=[1 6]; request input; cfg input; blank output size=[1 3]
function [gates,blank] = gate_deadtime(t,request,cfg)
%#codegen
% cfg = [enable, event grid, programmed deadtime]. Fall immediately;
% delay each rising edge. A pulse shorter than deadtime is suppressed.
persistent previous rise armed active
if isempty(previous)
 previous=zeros(1,6);rise=zeros(1,6);armed=false(1,6);active=zeros(1,6);
end
r=double(reshape(request,1,6)>0.5);gates=r;blank=zeros(1,3);
if cfg(1)==0,return;end
assert(all(r(1:2:5)+r(2:2:6)<=1));
tick=round(t/cfg(2));delay=round(cfg(3)/cfg(2));
for k=1:6
 if r(k)==0
  active(k)=0;armed(k)=false;
 elseif previous(k)==0
  rise(k)=tick;armed(k)=true;active(k)=0;
 end
 if armed(k)&&tick-rise(k)>=delay,active(k)=1;armed(k)=false;end
end
previous=r;gates=active;
assert(all(gates(1:2:5)+gates(2:2:6)<=1));
blank=1-gates(1:2:5)-gates(2:2:6);
end

== matlab function PMSM_FOC_R2026a/Universal Bridge/续流 ==
  settings: updateMethod=CONTINUOUS
  data: gates input; phase output size=[1 3]; state input; Vdc input; cfg input; diagnostic output size=[1 9]
function [phase,diagnostic] = bridge_freewheel(gates,state,Vdc,cfg)
%#codegen
% Static switched bridge for the present non-salient floating-star PMSM.
% cfg = [pole pairs, flux, zero-current band, drop enable, Ron, Vf].
% Positive current flows from pole to motor. During both-OFF, positive
% current uses the lower diode; negative current uses the upper diode.
x=reshape(state,1,4);g=reshape(gates,1,6);bus=max(Vdc,0);
theta=cfg(1)*x(4)+[0 -2*pi/3 2*pi/3];
current=x(1)*cos(theta)-x(2)*sin(theta);
emf=-cfg(1)*x(3)*cfg(2)*sin(theta);
pole=zeros(1,3);path=zeros(1,3);fixed=false(1,3);
ron=cfg(4)*cfg(5);vf=cfg(4)*cfg(6);
for k=1:3
 hi=g(2*k-1)>0.5;lo=g(2*k)>0.5;assert(~(hi&&lo));
 if hi,pole(k)=bus/2-ron*current(k);fixed(k)=true;
 elseif lo,pole(k)=-bus/2-ron*current(k);fixed(k)=true;
 elseif current(k)>cfg(3),pole(k)=-bus/2-vf;path(k)=-1;fixed(k)=true;
 elseif current(k)<-cfg(3),pole(k)=bus/2+vf;path(k)=1;fixed(k)=true;
 end
end
% Near zero, a disconnected phase follows its open-circuit EMF until a
% diode rail is reached. Small current band is a declared numerical model,
% not a device capacitance or exact diode complementarity solver.
neutral=0;
for pass=1:4
 count=sum(double(fixed));if count>0,neutral=sum((pole-emf).*double(fixed))/count;end
 changed=false;
 for k=1:3
  if ~fixed(k)
   pole(k)=emf(k)+neutral;
   if pole(k)>bus/2+vf,pole(k)=bus/2+vf;path(k)=1;fixed(k)=true;changed=true;
   elseif pole(k)<-bus/2-vf,pole(k)=-bus/2-vf;path(k)=-1;fixed(k)=true;changed=true;
   end
  end
 end
 if ~changed,break;end
end
% For near-zero open phases the neutral above enforces zero derivative;
% all fixed phases satisfy the usual floating-star mean subtraction.
phase=pole-sum(pole)/3;
diagnostic=[path pole current];
end

== matlab function PMSM_FOC_R2026a/限压/死区补偿 ==
  settings: updateMethod=DISCRETE  sampleTime=timing_control_sample
  data: current input; dq output size=[1 2]; theta input; Vdc input; cfg input; diagnostic output size=[1 8]
function [dq,diagnostic] = deadtime_comp(current,theta,Vdc,cfg)
%#codegen
% cfg = [enable, compensated deadtime, PWM period, current hysteresis].
% Uses measured current ONLY. Positive phase current needs positive voltage
% correction. Correction enters BEFORE the existing final dq circle limit.
persistent polarity
if isempty(polarity),polarity=zeros(1,3);end
dq=zeros(1,2);diagnostic=zeros(1,8);
if cfg(1)==0,return;end
i=reshape(current,1,3);
for k=1:3
 if i(k)>cfg(4),polarity(k)=1;
 elseif i(k)<-cfg(4),polarity(k)=-1;
 end
end
abc=max(Vdc,0)*cfg(2)/cfg(3)*polarity;abc=abc-sum(abc)/3;
alpha=(2*abc(1)-abc(2)-abc(3))/3;beta=(abc(2)-abc(3))/sqrt(3);
dq=[alpha*cos(theta)+beta*sin(theta),-alpha*sin(theta)+beta*cos(theta)];
diagnostic=[abc dq polarity];
end
